simulink model "Braccio_CtrlSimMdl_2025b"  (R2025b)
settings: Solver=ode1  StartTime=0.0  StopTime=inf  FixedStep=dt  RelTol=1e-3  EnableMultiTasking=on
values from neighbouring files (symbols this model uses):
  dt = 0.01    [Braccio_ini.m]    (also in Braccio_kinematics.m)
  jnt1 = rigidBodyJoint('jnt1','revolute')    [Braccio_ini.m]    (also in Braccio_kinematics.m)
  jnt2 = rigidBodyJoint('jnt2','revolute')    [Braccio_ini.m]    (also in Braccio_kinematics.m)
  jnt3 = rigidBodyJoint('jnt3','revolute')    [Braccio_ini.m]    (also in Braccio_kinematics.m)
  jnt4 = rigidBodyJoint('jnt4','revolute')    [Braccio_ini.m]    (also in Braccio_kinematics.m)
  jnt5 = rigidBodyJoint('jnt5','revolute')    [Braccio_ini.m]    (also in Braccio_kinematics.m)
undefined symbols (not defined in the file or in its folder): DiscIntNeverNeededParam, efence1_coord, Gripper, Pause, Run
libraries: sim3dlib x22, Braccio_lib x12, simulink x12, robotmaniplib x1, stm32f4xxblockslib x1, robotcorelib x1, robotsim3dlib x1
(part 2 of 2)

== matlab function Braccio_CtrlSimMdl_2025b/GripperVisu ==
  data: q_rad input; q_vis output size=13; q6 input; braccioGripper parameter
function q_vis = GripperVisu(q_rad, q6, braccioGripper)
%GRIPPERVISU Konfiguration fuer braccioRobotVis (Simulation 3D Robot)
%   q_rad   5x1 Gelenkwinkel q1..q5 [rad] (nach simpleDynamics)
%   q6      3x1 [q6 [rad]; Breite [m]; y-Mitte [m]] des gehaltenen Wuerfels
%           (q6_vis aus CubeInteraction, Breite 0 = kein Wuerfel)
%   q_vis  13x1 [q1..q5; Gelenke des Greifer-Mechanismus inkl. Federzinken]
q_vis = [q_rad(:); Braccio_gripperJoints(q6(1), braccioGripper, q6(2:3))];

== matlab function Braccio_CtrlSimMdl_2025b/CubeInteraction/SplitRows_pos ==
  data: v input; r1 output size=[1 3]; r2 output size=[1 3]; r3 output size=[1 3]; r4 output size=[1 3]; r5 output size=[1 3]; r6 output size=[1 3]
function [r1, r2, r3, r4, r5, r6] = SplitRows(v)
%SPLITROWS Zeilen 1x3 fuer die Vorrats-Actors cubeP1..cubeP6
%   v  3*nPool x 1, zeilenweise aneinandergehaengt (aus CubeGrasp)
M = reshape(v, 3, [])';
r1 = M(1, :);
r2 = M(2, :);
r3 = M(3, :);
r4 = M(4, :);
r5 = M(5, :);
r6 = M(6, :);

== matlab function Braccio_CtrlSimMdl_2025b/CubeInteraction/SplitRows_rot ==
  data: v input; r1 output size=[1 3]; r2 output size=[1 3]; r3 output size=[1 3]; r4 output size=[1 3]; r5 output size=[1 3]; r6 output size=[1 3]
function [r1, r2, r3, r4, r5, r6] = SplitRows(v)
%SPLITROWS Zeilen 1x3 fuer die Vorrats-Actors cubeP1..cubeP6
%   v  3*nPool x 1, zeilenweise aneinandergehaengt (aus CubeGrasp)
M = reshape(v, 3, [])';
r1 = M(1, :);
r2 = M(2, :);
r3 = M(3, :);
r4 = M(4, :);
r5 = M(5, :);
r6 = M(6, :);

== matlab function Braccio_CtrlSimMdl_2025b/CubeInteraction/SplitRows_color ==
  data: v input; r1 output size=[1 3]; r2 output size=[1 3]; r3 output size=[1 3]; r4 output size=[1 3]; r5 output size=[1 3]; r6 output size=[1 3]
function [r1, r2, r3, r4, r5, r6] = SplitRows(v)
%SPLITROWS Zeilen 1x3 fuer die Vorrats-Actors cubeP1..cubeP6
%   v  3*nPool x 1, zeilenweise aneinandergehaengt (aus CubeGrasp)
M = reshape(v, 3, [])';
r1 = M(1, :);
r2 = M(2, :);
r3 = M(3, :);
r4 = M(4, :);
r5 = M(5, :);
r6 = M(6, :);
